simulink library "lib_IC_GFM"  (R2026a)
settings: Solver=VariableStepAuto
undefined symbols (not defined in the file): block_buses, block_buses_DC, block_idx, block_toM, buses_lf, fb, fref, iC, invL, iR, iTf, Kic, Kiv, Kpc, Kpv, Nbuses_DC, omegab, op_intconv_GFM
libraries: simulink x4, sl_discontinuities x2
(part 1 of 2)
settings Model: Creator=atomas  LastModifiedBy=atomas

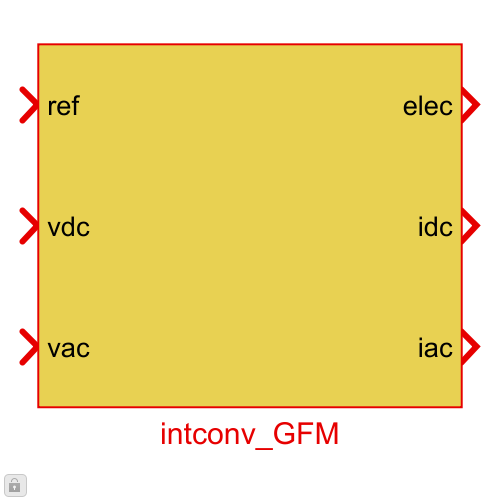
[thumbnail: Simulink's stored preview of the top-level diagram]
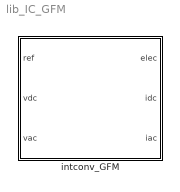
== system lib_IC_GFM ==
  intconv_GFM : Subsystem  mask(VCVSC){dynamic_VCC=Static, Lf=0.01, Rf=0.001, Rcf=1000000, Cfi=0.1, Kint=1, Tint=0.1, Bint=1, Kext=1, Bext=1, Text=0.1, Fi=1, Tf=0.01, mp=0.01, nq=0.01, VI_L=0.1, VI_R=0.01, WOF_Tf=0, L_out=0.1, R_out=0.01}
      mask prompts: dynamic_VCC "Dynamic behavior"; Lf "Filter inductance (pu)"; Rf "Filter resistance (pu)"; Rcf "Parallel resistance to C (pu)"; Cfi "Filter capacitance (pu)"; Fi "Current feedfordward gain"; Tf "Low-pass filter time constant (s)"; mp "Droop coefficient mp (pu)"; nq "Droop coefficient nq (pu)"; VI_L "Inductance (pu)"; VI_R "Resistance (pu)"; WOF_Tf "WOF time constant (s)"; L_out "Output inductance (p.u.)"; R_out "Output resistance (p.u.)"
      mask help: Grid-forming converter. VCC are the voltage and current controllers. Dynamic behavior includes the PI controllers, decoupling, current feedfordward and LC output filter. Static behavior consists of setting the reference voltage directly in the output. PC is the power controller including the droop control and low-pass filters for the power measurements.
      mask init:
      | [block_DC_buses, block_buses, block_DC_toM, block_toM, dparams, block_fref, block_idx, vcc_mode] = mask_init_intconv_GFM(gcb, dynamic_VCC);
      mask Help: web('Documentation/VCVSC.html')
      mask TypeOptions dynamic_VCC: Dynamic with limitation | Dynamic | Static | Dynamic VC and static CC
      mask TypeOptions Tf: PC/Tf
      mask TypeOptions mp: PC/mp
      mask TypeOptions nq: PC/nq
      mask TypeOptions VI_L: VI/L
      mask TypeOptions VI_R: VI/R
      mask TypeOptions WOF_Tf: VI/Tf
      mask DialogControl Container8 Prompt: Parameters
      mask DialogControl VCC Prompt: VCC
      mask DialogControl PC Prompt: PC
      mask DialogControl VI Prompt: VI
      mask DialogControl Container9 Prompt: Others

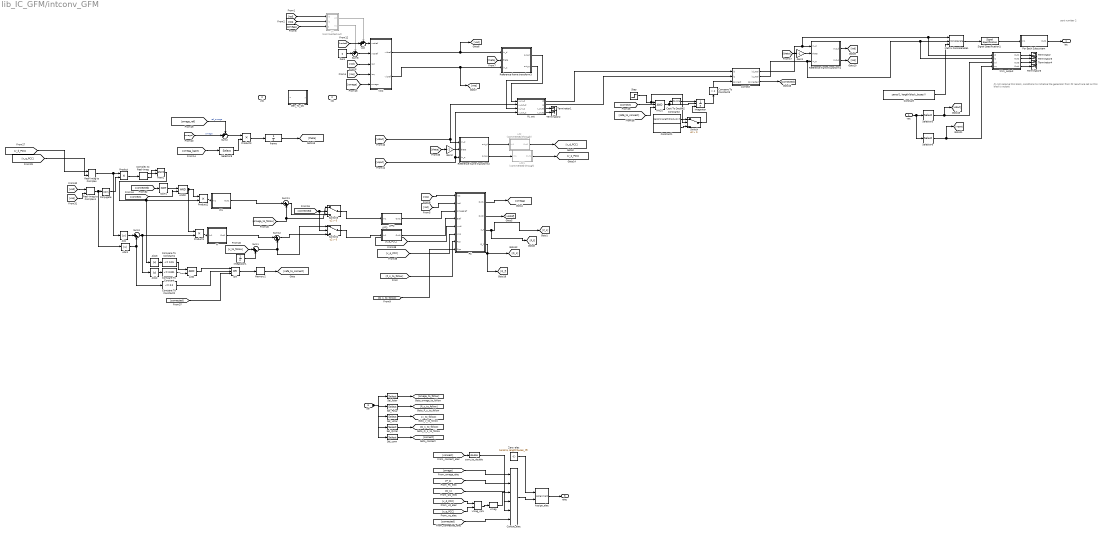
== system lib_IC_GFM/intconv_GFM ==
  note: port number 2
  note: do not rename this block, conditions to initialise the generator from PF result are set on this block's output
  vac : Inport
  vdc : Inport  Port=2
  ref : Inport  Port=3
  AND : Logic  IconShape=distinctive  AllPortsSameDT=off  OutDataTypeStr=boolean
  AND1 : Logic  Inputs=3  IconShape=distinctive  AllPortsSameDT=off  OutDataTypeStr=boolean
  AND2 : Logic  IconShape=distinctive  AllPortsSameDT=off  OutDataTypeStr=boolean
  Abs{,1..3} (4 alike) : Abs  ZeroCross=off  SaturateOnIntegerOverflow=off
  Assign_elec : Assignment  NumberOfDimensions=2  DiagnosticForDimensions=Warning  IndexOptions=Assign all,Index vector (dialog)  Indices=1,block_idx  OutputSizes=1
  Atan2 : Trigonometry  Operator=atan2
  Cast To Double2 : DataTypeConversion  OutDataTypeStr=double  SaturateOnIntegerOverflow=off  RndMeth=Floor
  Compare To Constant : simulink/Logic and Bit Operations/Compare To Constant  relop=<=  const=0.001  OutDataTypeStr=boolean  ZeroCross=off
  Compare To Constant1 : simulink/Logic and Bit Operations/Compare To Constant  relop=<=  const=0.01  OutDataTypeStr=boolean  ZeroCross=off
  Compare To Constant2 : simulink/Logic and Bit Operations/Compare To Constant  relop=<=  const=0.2  OutDataTypeStr=boolean  ZeroCross=off
  Compare To Constant3 : simulink/Logic and Bit Operations/Compare To Constant  relop=>  const=4  OutDataTypeStr=boolean  ZeroCross=off
  Complex to Real-Imag : ComplexToRealImag
  Concat_elec : Concatenate  NumInputs=6  Mode=Multidimensional array
  Conjugate : Math  Operator=conj  SignedPower=on  RndMeth=Zero
  Constant : Constant  Value=zeros(1, length(block_buses))  VectorParams1D=off
  Constant1 : Constant  Value=5*ones(1,length(block_idx))  VectorParams1D=off
  Constant2 : Constant  Value=zeros(1,length(block_idx))  VectorParams1D=off
  For Each Subsystem : Subsystem  TreatAsAtomicUnit=on
  Gain1 : Gain  Gain=-1
  Gain2 : Gain  Gain=-1
  Gen_To_DC : MATLAB Function  TreatAsAtomicUnit=on
  Integrator : Integrator  ExternalReset=falling  InitialConditionSource=external  InitialCondition=op_intconv_GFM.Integrator
  Integrator1 : Integrator  InitialCondition=op_intconv_GFM.Integrator1
  LPF : Subsystem  Commented=through
  LPF1 : Subsystem  Commented=through
  LPF2 : Subsystem
  LPF3 : Subsystem
  Matrix Concatenate1 : Concatenate  NumInputs=3  Mode=Multidimensional array
  Memory2 : Memory  InitialCondition=1
  NOT1 : Logic  Operator=NOT  IconShape=distinctive  AllPortsSameDT=off  OutDataTypeStr=boolean
  OR : Logic  Operator=OR  Inputs=3  IconShape=distinctive  AllPortsSameDT=off  OutDataTypeStr=boolean
  PC : Subsystem  mask(PC_VCVSC){Tf=Tf, mp=mp, nq=nq}
      mask prompts: Tf "Low-pass filter time constant (s)"; mp "Droop coefficient mp"; nq "Droop coefficient nq"
      mask help: Power controller of a grid-forming converter, including the droop control and low-pass filters for the power measurements.
      mask init:
      | [iTf, use_Tf] = mask_init_opt_filter(Tf);
  PI : Subsystem
  PI1 : Subsystem
  Product : Product
  Product1 : Product  OutDataTypeStr=double
  Product2 : Product  OutDataTypeStr=double
  Product3 : Product
  RL out : Subsystem  Variant=on  mask{dynamic=Dynamic, R=R_out, L=L_out, fbase=50}
      mask prompts: dynamic "Dynamic behavior"; R "Series resistance (p.u.)"; L "Inductance (p.u.)"; fbase "Base frequency (Hz)"
      mask init:
      | [invL, omegab, rl_mode] = mask_init_RL(dynamic, L, fbase);
      mask TypeOptions dynamic: Static | Dynamic | Static omega
  Real-Imag to Complex : RealImagToComplex
  Real-Imag to Complex1 : RealImagToComplex
  Reference frame transform1 : Subsystem
  Reference frame transform2 : Subsystem
  Reference frame transform3 : Subsystem
  Sel_Pstar : Selector  NumberOfDimensions=2  InputPortWidth=3  IndexOptions=Index vector (dialog),Index vector (dialog)  Indices=2,block_idx  OutputSizes=1
  Sel_Qstar : Selector  NumberOfDimensions=2  InputPortWidth=3  IndexOptions=Index vector (dialog),Index vector (dialog)  Indices=4,block_idx  OutputSizes=1
  Sel_conn : Selector  NumberOfDimensions=2  InputPortWidth=3  IndexOptions=Index vector (dialog),Index vector (dialog)  Indices=5,block_idx  OutputSizes=1
  Sel_fstar : Selector  NumberOfDimensions=2  InputPortWidth=3  IndexOptions=Index vector (dialog),Index vector (dialog)  Indices=1,block_idx  OutputSizes=1
  Sel_vstar : Selector  NumberOfDimensions=2  InputPortWidth=3  IndexOptions=Index vector (dialog),Index vector (dialog)  Indices=3,block_idx  OutputSizes=1
  Selector5 : Selector  NumberOfDimensions=2  InputPortWidth=3  IndexOptions=Index vector (dialog),Index vector (dialog)  Indices=1,block_buses  OutputSizes=1,1
  Selector6 : Selector  NumberOfDimensions=2  InputPortWidth=3  IndexOptions=Index vector (dialog),Index vector (dialog)  Indices=2,block_buses  OutputSizes=1,1
  Selector8 : Selector  InputPortWidth=length(fref.ref_units)  IndexOptions=Index vector (dialog)  Indices=block_fref  OutputSizes=1
  Signal Specification1 : SignalSpecification  Dimensions=[3 length(block_buses)]
  Step : Step  Time=0.01  SampleTime=0  VectorParams1D=off  ZeroCross=off
  Sum1 : Sum  Inputs=|++
  Sum11 : Sum  Inputs=|++
  Sum12 : Sum  Inputs=|++
  Sum2 : Sum  Inputs=-+|
  Sum3 : Sum  Inputs=|+-
  Sum8 : Sum  Inputs=++|
  Switch : Switch  Criteria=u2 > Threshold  SaturateOnIntegerOverflow=off  InputSameDT=off
  Switch2 : Switch  Criteria=u2 > Threshold  SaturateOnIntegerOverflow=off  InputSameDT=off
  Switch3 : Switch  Criteria=u2 > Threshold  SaturateOnIntegerOverflow=off  InputSameDT=off
  Terminator{,1..5} (6 alike) : Terminator
  VCC : Subsystem  Variant=on
  VI : Subsystem  Commented=on  mask{L=VI_L, R=VI_R, Tf=WOF_Tf}
      mask prompts: L "Inductance (pu)"; R "Resistance (pu)"; Tf "WOF time constant (s)"
      mask init:
      | [iTf, use_Tf] = mask_init_opt_filter(Tf);
  Zero : Constant  Value=0  OutDataTypeStr=Inherit: Inherit via back propagation
  Zero_elec : Constant  Value=zeros(6, length(buses_lf))
  conn_to_double : DataTypeConversion  OutDataTypeStr=double  SaturateOnIntegerOverflow=off  RndMeth=Floor
  connect : Subsystem
  frame : Integrator  InitialCondition=op_intconv_GFM.frame  IgnoreLimit=on
  trim_output : Subsystem
  vmag : ComplexToMagnitudeAngle  Output=Magnitude
  vmag_cplx : RealImagToComplex
  vod : Sum  Inputs=++|
  iac : Outport
  idc : Outport  Port=2
  elec : Outport  Port=3
  wires:
  LPF3/1(Out1) -> PC/4(Eref)
  LPF2/1(Out1) -> PC/3(omegaref)
  [connect] -> AND2/2
  Compare To Constant3/1 -> connect/3(connect)
  Integrator1/1 -> Sum1/2
  [v_to_follow] -> Sum1/1
  [Q_s_to_follow] -> PC/8(Qsp)
  [P_s_to_follow] -> PC/7(Psp)
  Switch2/1 -> LPF3/1(In1)
  Switch3/1 -> LPF2/1(In1)
  Sum11/1 -> Switch3/3
  PI1/1(Out1) -> Sum11/1
  PI/1(Out1) -> Sum12/1
  [connected] -> Switch3/2, Switch2/2
  [omega_to_follow] -> Switch3/1, Sum11/2
  Sum1/1 -> Sum12/2, Switch2/1
  Sum12/1 -> Switch2/3
  VCC/2(viqref) -> Reference frame transform3/3(in_q), [voq]
  VCC/1(vidref) -> Reference frame transform3/1(in_d), [vod]
  Switch/1 -> Integrator/3
  Cast To Double2/1 -> Integrator/1
  AND1/1 -> Integrator/2, Cast To Double2/1
  [safe_to_connect] -> AND1/3
  Constant1/1 -> Switch/3
  Step/1 -> AND1/1, Switch/2
  Constant2/1 -> Switch/1
  Integrator/1 -> Compare To Constant3/1
  [connect] -> AND1/2
  AND2/1 -> Product2/1, Product1/1
  [connected] -> NOT1/1
  NOT1/1 -> AND2/1
  Selector5/1 -> trim_output/3(vd), [vdout]
  Selector6/1 -> trim_output/4(vq), [vqout]
  vac/1 -> Selector5/1, Selector6/1
  trim_output/4(Out4) -> Terminator5/1
  trim_output/3(Out3) -> Terminator4/1
  trim_output/2(Out2) -> Terminator3/1
  trim_output/1(Out1) -> Terminator/1
  [v_q_PCC] -> PC/6(voq)
  [v_d_PCC] -> PC/5(vodi)
  Signal Specification1/1 -> For Each Subsystem/1(In1)
  For Each Subsystem/1(Out1) -> iac/1
  Constant/1 -> Matrix Concatenate1/3
  Matrix Concatenate1/1 -> Signal Specification1/1
  [vdout] -> Reference frame transform2/1(in_d), RL out/2(v_out_d)
  LPF1/1(Out1) -> [v_q_PCC]
  LPF/1(Out1) -> [v_d_PCC]
  [vqout] -> RL out/4(v_out_q), Reference frame transform2/3(in_q)
  Memory2/1 -> [safe_to_connect]
  [connected] -> OR/3
  Compare To Constant2/1 -> OR/2
  OR/1 -> Memory2/1
  AND/1 -> OR/1
  Compare To Constant1/1 -> AND/1
  Abs3/1 -> Compare To Constant1/1
  Compare To Constant/1 -> AND/2
  Abs2/1 -> Compare To Constant/1
  Abs1/1 -> Sum3/2, Compare To Constant2/1
  Atan2/1 -> Product2/2, Abs3/1
  Product2/1 -> PI1/1(In1)
  Product1/1 -> PI/1(In1)
  Sum3/1 -> Product1/2, Abs2/1
  Abs/1 -> Sum3/1
  Complex to Real-Imag/1 -> Atan2/2
  Complex to Real-Imag/2 -> Atan2/1
  Product/1 -> Complex to Real-Imag/1
  Conjugate/1 -> Product/2
  Real-Imag to Complex/1 -> Product/1, Abs/1
  Real-Imag to Complex1/1 -> Conjugate/1, Abs1/1
  [voq] -> Real-Imag to Complex1/2
  [vod] -> Real-Imag to Complex1/1
  [v_q_PCC] -> Real-Imag to Complex/2
  [v_d_PCC] -> Real-Imag to Complex/1
  Reference frame transform2/2(out_q) -> LPF1/1(In1)
  Reference frame transform2/1(out_d) -> LPF/1(In1)
  RL out/4(v_outq) -> Terminator2/1
  RL out/3(v_outd) -> Terminator1/1
  connect/2(iq_real) -> Reference frame transform1/3(in_q), Matrix Concatenate1/2, trim_output/2(iq)
  connect/1(id_real) -> Reference frame transform1/1(in_d), Matrix Concatenate1/1, trim_output/1(id)
  VI/2(vq) -> Sum8/1
  VI/1(vd) -> vod/1
  Reference frame transform1/1(out_d) -> [iod]
  RL out/2(iq) -> connect/2(iq)
  Reference frame transform3/2(out_q) -> RL out/3(v_in_q)
  Reference frame transform3/1(out_d) -> RL out/1(v_in_d)
  Reference frame transform1/2(out_q) -> [ioq]
  [ioq] -> PC/1(ioq)
  [iod] -> PC/2(iodi)
  PC/2(Out2) -> [vodref]
  PC/1(Out1) -> [omega]
  [theta] -> Reference frame transform3/2(theta)
  [omega] -> VCC/5(omega)
  [vodref] -> vod/2
  Zero/1 -> Sum8/2
  [iod] -> VCC/3(iod)
  [ioq] -> VCC/4(ioq)
  Gain1/1 -> Reference frame transform1/2(theta)
  [theta] -> Gain1/1
  RL out/1(id) -> connect/1(id)
  Sum2/1 -> Product3/1
  [omega_ref] -> Sum2/1  "ref_omega"
  [omega] -> Sum2/2  "omega"
  connect/3(connected) -> [connected]
  PC/3(P_f) -> [P_f], [P_s]
  PC/4(Q_f) -> [Q_f], [Q_s]
  frame/1 -> [theta]
  Product3/1 -> frame/1
  [theta] -> Gain2/1
  Gain2/1 -> Reference frame transform2/2(theta)
  [iod] -> VI/1(id)
  [ioq] -> VI/2(iq)
  [omega] -> VI/3(omega)
  vod/1 -> VCC/1(vodref)
  Sum8/1 -> VCC/2(voqref)
  Selector8/1 -> Product3/2
  [omega_base] -> Selector8/1
  ref/1 -> Sel_fstar/1, Sel_Pstar/1, Sel_vstar/1, Sel_Qstar/1, Sel_conn/1
  Sel_fstar/1 -> [omega_to_follow]
  Sel_Pstar/1 -> [P_s_to_follow]
  Sel_vstar/1 -> [v_to_follow]
  Sel_Qstar/1 -> [Q_s_to_follow]
  Sel_conn/1 -> [connect]
  [connect] -> conn_to_double/1
  [v_d_PCC] -> vmag_cplx/1
  [v_q_PCC] -> vmag_cplx/2
  vmag_cplx/1 -> vmag/1
  [omega] -> Concat_elec/1
  [P_s] -> Concat_elec/2
  vmag/1 -> Concat_elec/3
  [Q_s] -> Concat_elec/4
  conn_to_double/1 -> Concat_elec/5
  [connected] -> Concat_elec/6
  Zero_elec/1 -> Assign_elec/1
  Concat_elec/1 -> Assign_elec/2
  Assign_elec/1 -> elec/1

== system lib_IC_GFM/intconv_GFM/For Each Subsystem ==
  In1 : Inport  Partition=on  PartitionDimension=1  PartitionWidth=1  PartitionOffset=0
  For Each : ForEach  DisableCoverage=on
  State-Space : StateSpace  A=[]  B=[]  C=[]  D=block_toM  InitialCondition=0  ParameterTunability=Optimized
  Transpose : Math  Operator=transpose
  Transpose1 : Math  Operator=transpose
  Out1 : Outport  ConcatenationDimension=1
  wires:
  In1/1 -> Transpose/1
  Transpose1/1 -> Out1/1
  Transpose/1 -> State-Space/1
  State-Space/1 -> Transpose1/1

== system lib_IC_GFM/intconv_GFM/LPF ==
  In1 : Inport
  Gain : Gain  Gain=1e2
  I : Integrator  InitialCondition=op_intconv_GFM.LPF_I
  Sum4 : Sum  Inputs=|+-
  Out1 : Outport
  wires:
  I/1 -> Sum4/2, Out1/1
  In1/1 -> Sum4/1
  Sum4/1 -> Gain/1
  Gain/1 -> I/1

== system lib_IC_GFM/intconv_GFM/LPF1 ==
  In1 : Inport
  Gain : Gain  Gain=1e2
  I : Integrator  InitialCondition=op_intconv_GFM.LPF1_I
  Sum4 : Sum  Inputs=|+-
  Out1 : Outport
  wires:
  Gain/1 -> I/1
  Sum4/1 -> Gain/1
  In1/1 -> Sum4/1
  I/1 -> Out1/1, Sum4/2

== system lib_IC_GFM/intconv_GFM/LPF2 ==
  In1 : Inport
  Gain : Gain  Gain=1e2
  I : Integrator  InitialCondition=op_intconv_GFM.LPF2_I
  Sum4 : Sum  Inputs=|+-
  Out1 : Outport
  wires:
  Gain/1 -> I/1
  Sum4/1 -> Gain/1
  In1/1 -> Sum4/1
  I/1 -> Out1/1, Sum4/2

== system lib_IC_GFM/intconv_GFM/LPF3 ==
  In1 : Inport
  Gain : Gain  Gain=1e2
  I : Integrator  InitialCondition=op_intconv_GFM.LPF3_I
  Sum4 : Sum  Inputs=|+-
  Out1 : Outport
  wires:
  I/1 -> Sum4/2, Out1/1
  In1/1 -> Sum4/1
  Sum4/1 -> Gain/1
  Gain/1 -> I/1

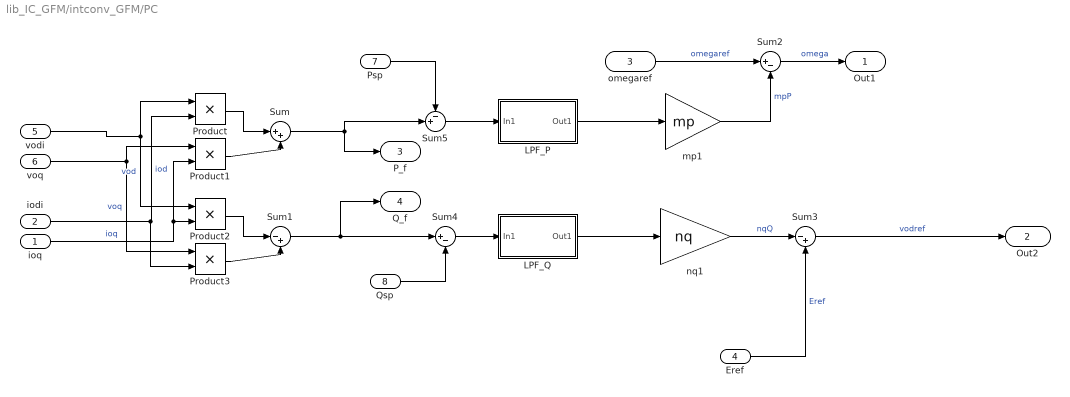
== system lib_IC_GFM/intconv_GFM/PC ==
  ioq : Inport
  iodi : Inport  Port=2
  omegaref : Inport  Port=3
  Eref : Inport  Port=4
  vodi : Inport  Port=5
  voq : Inport  Port=6
  Psp : Inport  Port=7
  Qsp : Inport  Port=8
  LPF_P : Subsystem  Variant=on
  LPF_Q : Subsystem  Variant=on
  Product{,1..3} (4 alike) : Product
  Sum : Sum  Inputs=|++
  Sum1 : Sum  Inputs=|-+
  Sum2 : Sum  Inputs=|+-
  Sum3 : Sum  Inputs=|-+
  Sum4 : Sum  Inputs=|+-
  Sum5 : Sum  Inputs=-+|
  mp1 : Gain  Gain=mp
  nq1 : Gain  Gain=nq
  Out1 : Outport
  Out2 : Outport  Port=2
  P_f : Outport  Port=3
  Q_f : Outport  Port=4
  wires:
  LPF_Q/1(Out1) -> nq1/1
  Sum4/1 -> LPF_Q/1(In1)
  LPF_P/1(Out1) -> mp1/1
  Sum5/1 -> LPF_P/1(In1)
  Sum3/1 -> Out2/1  "vodref"
  Psp/1 -> Sum5/1
  Qsp/1 -> Sum4/2
  ioq/1 -> Product1/2, Product2/2  "ioq"
  iodi/1 -> Product/2, Product3/2  "iod"
  voq/1 -> Product3/1, Product1/1  "voq"
  mp1/1 -> Sum2/2  "mpP"
  Sum1/1 -> Sum4/1, Q_f/1
  Sum/1 -> P_f/1, Sum5/2
  omegaref/1 -> Sum2/1  "omegaref"
  Eref/1 -> Sum3/2  "Eref"
  nq1/1 -> Sum3/1  "nqQ"
  Product3/1 -> Sum1/2
  Product2/1 -> Sum1/1
  Product1/1 -> Sum/2
  Product/1 -> Sum/1
  vodi/1 -> Product/1, Product2/1  "vod"
  Sum2/1 -> Out1/1  "omega"

== system lib_IC_GFM/intconv_GFM/PI ==
  In1 : Inport
  Gain : Gain  Gain=0.1
  Gain1 : Gain  Gain=0.2
  I : Integrator  InitialCondition=op_intconv_GFM.PI_I
  Sum10 : Sum  Inputs=|++
  Out1 : Outport
  wires:
  In1/1 -> Gain1/1, Gain/1
  Sum10/1 -> Out1/1
  Gain/1 -> Sum10/1
  I/1 -> Sum10/2
  Gain1/1 -> I/1

== system lib_IC_GFM/intconv_GFM/PI1 ==
  In1 : Inport
  Gain : Gain  Gain=0.1/100/pi
  Gain1 : Gain  Gain=0.2/100/pi
  I : Integrator  InitialCondition=op_intconv_GFM.PI1_I
  Sum10 : Sum  Inputs=|++
  Out1 : Outport
  wires:
  Gain1/1 -> I/1
  I/1 -> Sum10/2
  Gain/1 -> Sum10/1
  Sum10/1 -> Out1/1
  In1/1 -> Gain/1, Gain1/1

== system lib_IC_GFM/intconv_GFM/RL out ==
  note: 1) Add Subsystem or Model blocks as valid variant choices.
      | 2) You cannot connect blocks at this level. At simulation, connectivity is automatically
      | determined, based on the active variant and port name matching.
  v_in_d : Inport
  v_out_d : Inport  Port=2
  v_in_q : Inport  Port=3
  v_out_q : Inport  Port=4
  dynamic : Subsystem  VariantControl=rl_mode == 1
  static : Subsystem  VariantControl=rl_mode == 2
  static_omega : Subsystem  VariantControl=(default)
  id : Outport
  iq : Outport  Port=2
  v_outd : Outport  Port=3
  v_outq : Outport  Port=4

== system lib_IC_GFM/intconv_GFM/Reference frame transform1 ==
  in_d : Inport
  theta : Inport  Port=2
  in_q : Inport  Port=3
  Complex to Real-Imag : ComplexToRealImag
  Cos : Trigonometry  SCDEnableBlockLinearizationSpecification=on  Operator=cos
  Product : Product
  Real-Imag to Complex : RealImagToComplex
  Real-Imag to Complex1 : RealImagToComplex
  Sin : Trigonometry  SCDEnableBlockLinearizationSpecification=on
  out_d : Outport
  out_q : Outport  Port=2
  wires:
  in_d/1 -> Real-Imag to Complex/1
  in_q/1 -> Real-Imag to Complex/2
  Complex to Real-Imag/1 -> out_d/1
  Sin/1 -> Real-Imag to Complex1/2
  Cos/1 -> Real-Imag to Complex1/1
  theta/1 -> Cos/1, Sin/1
  Product/1 -> Complex to Real-Imag/1
  Real-Imag to Complex/1 -> Product/2
  Real-Imag to Complex1/1 -> Product/1
  Complex to Real-Imag/2 -> out_q/1

== system lib_IC_GFM/intconv_GFM/Reference frame transform2 ==
  in_d : Inport
  theta : Inport  Port=2
  in_q : Inport  Port=3
  Complex to Real-Imag : ComplexToRealImag
  Cos : Trigonometry  SCDEnableBlockLinearizationSpecification=on  Operator=cos
  Product : Product
  Real-Imag to Complex : RealImagToComplex
  Real-Imag to Complex1 : RealImagToComplex
  Sin : Trigonometry  SCDEnableBlockLinearizationSpecification=on
  out_d : Outport
  out_q : Outport  Port=2
  wires:
  Complex to Real-Imag/2 -> out_q/1
  Real-Imag to Complex1/1 -> Product/1
  Real-Imag to Complex/1 -> Product/2
  Product/1 -> Complex to Real-Imag/1
  theta/1 -> Sin/1, Cos/1
  Cos/1 -> Real-Imag to Complex1/1
  Sin/1 -> Real-Imag to Complex1/2
  Complex to Real-Imag/1 -> out_d/1
  in_q/1 -> Real-Imag to Complex/2
  in_d/1 -> Real-Imag to Complex/1

== system lib_IC_GFM/intconv_GFM/Reference frame transform3 ==
  in_d : Inport
  theta : Inport  Port=2
  in_q : Inport  Port=3
  Complex to Real-Imag : ComplexToRealImag
  Cos : Trigonometry  SCDEnableBlockLinearizationSpecification=on  Operator=cos
  Product : Product
  Real-Imag to Complex : RealImagToComplex
  Real-Imag to Complex1 : RealImagToComplex
  Sin : Trigonometry  SCDEnableBlockLinearizationSpecification=on
  out_d : Outport
  out_q : Outport  Port=2
  wires:
  in_d/1 -> Real-Imag to Complex/1
  in_q/1 -> Real-Imag to Complex/2
  Complex to Real-Imag/1 -> out_d/1
  Sin/1 -> Real-Imag to Complex1/2
  Cos/1 -> Real-Imag to Complex1/1
  theta/1 -> Sin/1, Cos/1
  Product/1 -> Complex to Real-Imag/1
  Real-Imag to Complex/1 -> Product/2
  Real-Imag to Complex1/1 -> Product/1
  Complex to Real-Imag/2 -> out_q/1

== system lib_IC_GFM/intconv_GFM/VCC ==
  note: 1) Add Subsystem or Model blocks as valid variant choices.
      | 2) You cannot connect blocks at this level. At simulation, connectivity is automatically
      | determined, based on the active variant and port name matching.
  vodref : Inport
  voqref : Inport  Port=2
  iod : Inport  Port=3
  ioq : Inport  Port=4
  omega : Inport  Port=5
  dynamic : Subsystem  VariantControl=vcc_mode == 1
  dynamic_VC : Subsystem  VariantControl=vcc_mode == 3
  dynamic_limiting : Subsystem  VariantControl=vcc_mode == 2
  static : Subsystem  VariantControl=(default)
  vidref : Outport
  viqref : Outport  Port=2

== system lib_IC_GFM/intconv_GFM/VI ==
  id : Inport
  iq : Inport  Port=2
  omega : Inport  Port=3
  Gain : Gain  Gain=L
  Gain1 : Gain  Gain=R
  Gain2 : Gain  Gain=L
  Gain3 : Gain  Gain=R
  Product : Product
  Product1 : Product
  Sum : Sum  Inputs=-+|
  Sum1 : Sum  Inputs=|--
  WOF_d : Subsystem  Variant=on
  WOF_q : Subsystem  Variant=on
  vd : Outport
  vq : Outport  Port=2
  wires:
  WOF_q/1(Out1) -> Gain3/1, Gain/1
  iq/1 -> WOF_q/1(In1)
  WOF_d/1(Out1) -> Gain2/1, Gain1/1
  id/1 -> WOF_d/1(In1)
  Gain/1 -> Product/1
  omega/1 -> Product/2, Product1/1
  Product/1 -> Sum/2
  Gain2/1 -> Product1/2
  Product1/1 -> Sum1/1
  Gain1/1 -> Sum/1
  Gain3/1 -> Sum1/2
  Sum/1 -> vd/1
  Sum1/1 -> vq/1

== system lib_IC_GFM/intconv_GFM/connect ==
  id : Inport
  iq : Inport  Port=2
  connect : Inport  Port=3
  Switch : Switch  Criteria=u2 > Threshold  ZeroCross=off  SaturateOnIntegerOverflow=off  InputSameDT=off
  Switch1 : Switch  Criteria=u2 > Threshold  ZeroCross=off  SaturateOnIntegerOverflow=off  InputSameDT=off
  Zero1 : Constant  Value=0  VectorParams1D=off  OutDataTypeStr=Inherit: Inherit via back propagation
  Zero2 : Constant  Value=0  VectorParams1D=off  OutDataTypeStr=Inherit: Inherit via back propagation
  id_real : Outport
  iq_real : Outport  Port=2
  connected : Outport  Port=3  OutDataTypeStr=boolean
  wires:
  Zero2/1 -> Switch1/3
  iq/1 -> Switch1/1
  Switch1/1 -> iq_real/1
  connect/1 -> Switch/2, Switch1/2, connected/1
  id/1 -> Switch/1
  Zero1/1 -> Switch/3
  Switch/1 -> id_real/1

== system lib_IC_GFM/intconv_GFM/trim_output ==
  id : Inport
  iq : Inport  Port=2
  vd : Inport  Port=3
  vq : Inport  Port=4
  Out1 : Outport
  Out2 : Outport  Port=2
  Out3 : Outport  Port=3
  Out4 : Outport  Port=4
  wires:
  iq/1 -> Out2/1
  vd/1 -> Out3/1
  vq/1 -> Out4/1
  id/1 -> Out1/1

== system lib_IC_GFM/intconv_GFM/PC/LPF_P ==
  note: 1) Add Subsystem or Model blocks as valid variant choices.
      | 2) You cannot connect blocks at this level. At simulation, connectivity is automatically
      | determined, based on the active variant and port name matching.
  In1 : Inport
  Active : Subsystem  VariantControl=use_Tf == 1
  Bypass : Subsystem  VariantControl=(default)
  Out1 : Outport

== system lib_IC_GFM/intconv_GFM/PC/LPF_Q ==
  note: 1) Add Subsystem or Model blocks as valid variant choices.
      | 2) You cannot connect blocks at this level. At simulation, connectivity is automatically
      | determined, based on the active variant and port name matching.
  In1 : Inport
  Active : Subsystem  VariantControl=use_Tf == 1
  Bypass : Subsystem  VariantControl=(default)
  Out1 : Outport

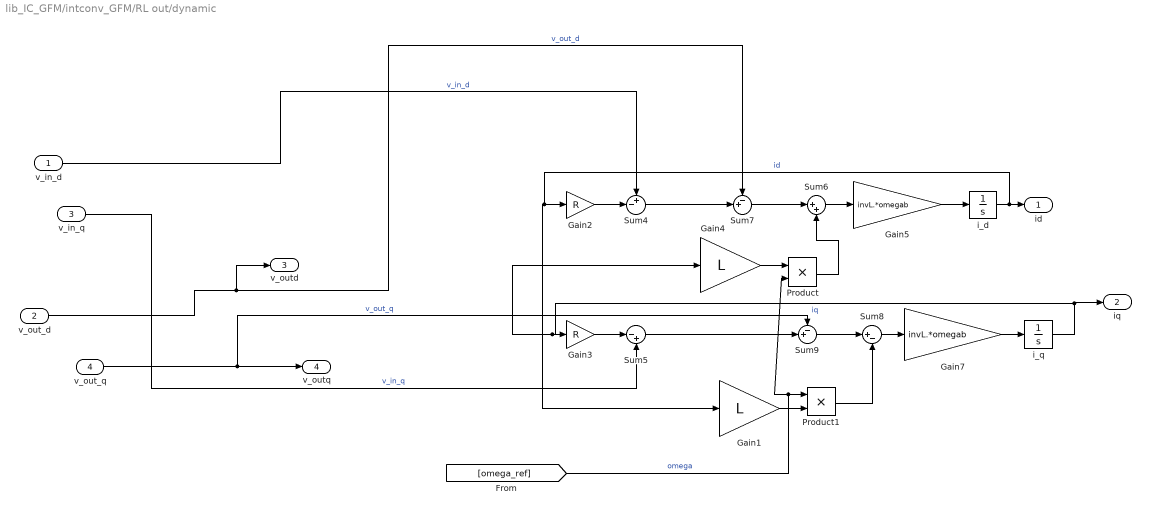
== system lib_IC_GFM/intconv_GFM/RL out/dynamic ==
  v_in_d : Inport
  v_out_d : Inport  Port=2
  v_in_q : Inport  Port=3
  v_out_q : Inport  Port=4
  Gain1 : Gain  Gain=L
  Gain2 : Gain  Gain=R
  Gain3 : Gain  Gain=R
  Gain4 : Gain  Gain=L
  Gain5 : Gain  Gain=invL.*omegab
  Gain7 : Gain  Gain=invL.*omegab
  Product : Product
  Product1 : Product
  Sum4 : Sum  Inputs=+-|
  Sum5 : Sum  Inputs=|-+
  Sum6 : Sum  Inputs=|++
  Sum7 : Sum  Inputs=-+|
  Sum8 : Sum  Inputs=|+-
  Sum9 : Sum  Inputs=-+|
  i_d : Integrator  InitialCondition=op_intconv_GFM.RL_out_dynamic_i_d
  i_q : Integrator  InitialCondition=op_intconv_GFM.RL_out_dynamic_i_q
  id : Outport
  iq : Outport  Port=2
  v_outd : Outport  Port=3
  v_outq : Outport  Port=4
  wires:
  v_in_q/1 -> Sum5/2  "v_in_q"
  v_in_d/1 -> Sum4/1  "v_in_d"
  Gain2/1 -> Sum4/2
  i_d/1 -> Gain2/1, Gain1/1, id/1  "id"
  Sum6/1 -> Gain5/1
  [omega_ref] -> Product1/1, Product/2  "omega"
  Gain5/1 -> i_d/1
  Product/1 -> Sum6/2
  Sum8/1 -> Gain7/1
  Sum4/1 -> Sum7/2
  Product1/1 -> Sum8/2
  Gain4/1 -> Product/1
  Sum7/1 -> Sum6/1
  Gain3/1 -> Sum5/1
  Sum5/1 -> Sum9/2
  Gain7/1 -> i_q/1
  i_q/1 -> Gain3/1, Gain4/1, iq/1  "iq"
  Gain1/1 -> Product1/2
  Sum9/1 -> Sum8/1
  v_out_d/1 -> Sum7/1, v_outd/1  "v_out_d"
  v_out_q/1 -> Sum9/1, v_outq/1  "v_out_q"

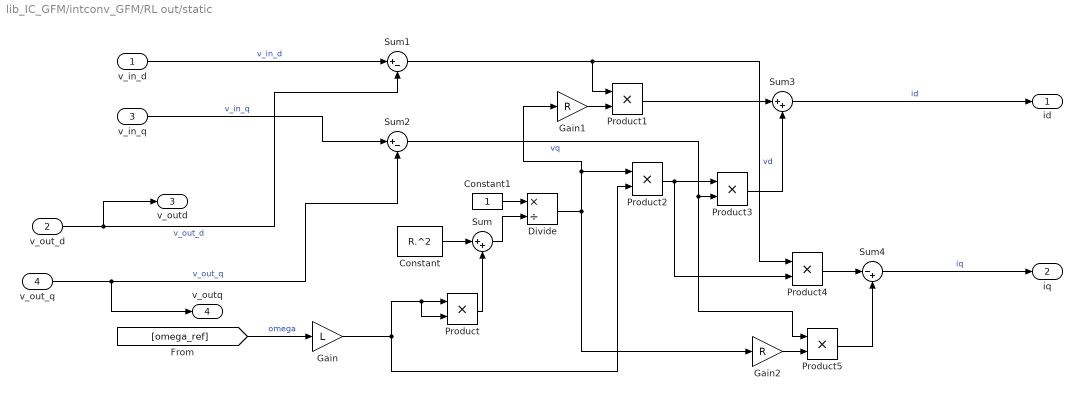
== system lib_IC_GFM/intconv_GFM/RL out/static ==
  v_in_d : Inport
  v_out_d : Inport  Port=2
  v_in_q : Inport  Port=3
  v_out_q : Inport  Port=4
  Constant : Constant  Value=R.^2
  Constant1 : Constant
  Divide : Product  Inputs=*/
  Gain : Gain  Gain=L
  Gain1 : Gain  Gain=R
  Gain2 : Gain  Gain=R
  Product{,1..5} (6 alike) : Product
  Sum : Sum  Inputs=|++
  Sum1 : Sum  Inputs=|+-
  Sum2 : Sum  Inputs=|+-
  Sum3 : Sum  Inputs=|++
  Sum4 : Sum  Inputs=|-+
  id : Outport
  iq : Outport  Port=2
  v_outd : Outport  Port=3
  v_outq : Outport  Port=4
  wires:
  v_in_q/1 -> Sum2/1  "v_in_q"
  v_out_d/1 -> Sum1/2, v_outd/1  "v_out_d"
  Sum/1 -> Divide/2
  Gain2/1 -> Product5/2
  Product/1 -> Sum/2
  Product1/1 -> Sum3/1
  Product5/1 -> Sum4/2
  Constant/1 -> Sum/1
  Sum2/1 -> Product3/2, Product5/1  "vq"
  Gain/1 -> Product2/2, Product/1, Product/2
  Constant1/1 -> Divide/1
  Product3/1 -> Sum3/2
  Sum1/1 -> Product4/1, Product1/1  "vd"
  Divide/1 -> Product2/1, Gain1/1, Gain2/1
  Product4/1 -> Sum4/1
  Product2/1 -> Product3/1, Product4/2
  Gain1/1 -> Product1/2
  Sum3/1 -> id/1  "id"
  Sum4/1 -> iq/1  "iq"
  v_out_q/1 -> Sum2/2, v_outq/1  "v_out_q"
  v_in_d/1 -> Sum1/1  "v_in_d"
  [omega_ref] -> Gain/1  "omega"

== system lib_IC_GFM/intconv_GFM/RL out/static_omega ==
  v_in_d : Inport
  v_out_d : Inport  Port=2
  v_in_q : Inport  Port=3
  v_out_q : Inport  Port=4
  Gain : Gain  Gain=1./(R.^2+L.^2)
  Gain2 : Gain  Gain=1./(R.^2+L.^2)
  Gain3 : Gain  Gain=R
  Gain4 : Gain  Gain=L
  Gain5 : Gain  Gain=L
  Gain6 : Gain  Gain=R
  Sum : Sum  Inputs=|++
  Sum1 : Sum  Inputs=|+-
  Sum2 : Sum  Inputs=|+-
  Sum3 : Sum  Inputs=|-+
  id : Outport
  iq : Outport  Port=2
  v_outd : Outport  Port=3
  v_outq : Outport  Port=4
  wires:
  Gain6/1 -> Sum3/2
  Sum3/1 -> iq/1
  Gain5/1 -> Sum3/1
  Sum/1 -> id/1
  Gain2/1 -> Gain4/1, Gain6/1
  Gain4/1 -> Sum/2
  Gain3/1 -> Sum/1
  Gain/1 -> Gain3/1, Gain5/1
  Sum2/1 -> Gain2/1  "vq"
  Sum1/1 -> Gain/1  "vd"
  v_out_d/1 -> Sum1/2, v_outd/1  "v_out_d"
  v_out_q/1 -> Sum2/2, v_outq/1  "v_out_q"
  v_in_d/1 -> Sum1/1  "v_in_d"
  v_in_q/1 -> Sum2/1  "v_in_q"

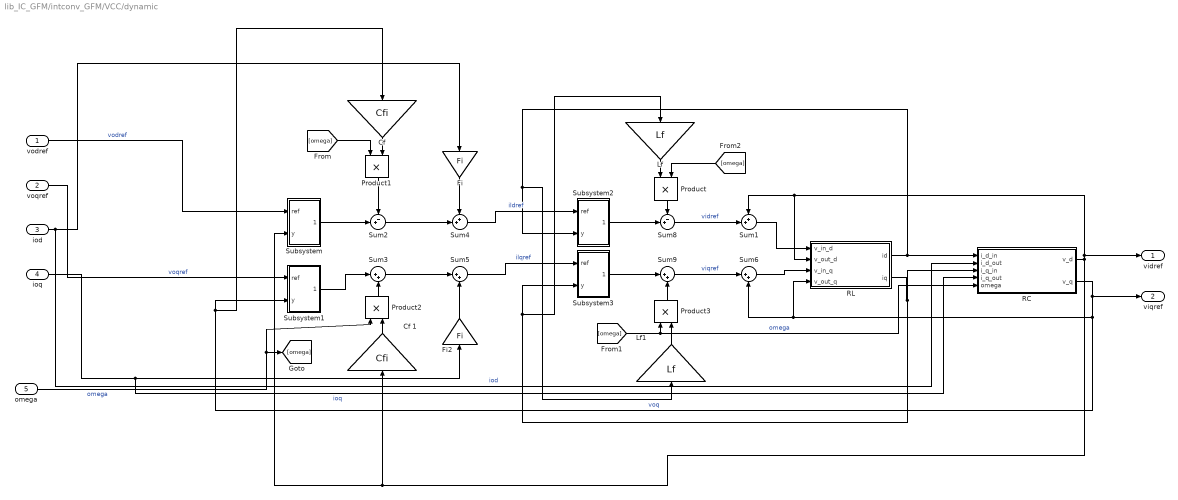
== system lib_IC_GFM/intconv_GFM/VCC/dynamic ==
  vodref : Inport
  voqref : Inport  Port=2
  iod : Inport  Port=3
  ioq : Inport  Port=4
  omega : Inport  Port=5
  Cf : Gain  Gain=Cfi
  Cf 1 : Gain  Gain=Cfi
  Fi : Gain  Gain=Fi
  Fi2 : Gain  Gain=Fi
  "Lf " : Gain  Gain=Lf
  Lf1 : Gain  Gain=Lf
  Product{,1..3} (4 alike) : Product
  RC : Subsystem  Variant=on  mask{dynamic=Dynamic, R=Rcf, C=Cfi, fbase=50}
      mask prompts: dynamic "Dynamic behavior"; R "Parallel resistance (p.u.)"; C "Capacitance (p.u.)"; fbase "Base frequency (Hz)"
      mask init:
      | [iC, iR, omegab, rc_mode] = mask_init_RC(dynamic, R, C, fbase);
      mask TypeOptions dynamic: Dynamic | Static | Static omega
  RL : Subsystem  Variant=on  mask(Line){dynamic=Dynamic, R=Rf, L=Lf, fbase=fb}
      mask prompts: dynamic "Dynamic behavior"; R "Series resistance (p.u.)"; L "Inductance (p.u.)"; fbase "Base frequency (Hz)"
      mask init:
      | [invL, omegab, rl_mode] = mask_init_RL(dynamic, L, fbase);
      mask Help: web('Documentation/RL.html')
      mask TypeOptions dynamic: Static | Dynamic | Static omega
  Subsystem : Subsystem
  Subsystem1 : Subsystem
  Subsystem2 : Subsystem
  Subsystem3 : Subsystem
  Sum1 : Sum  Inputs=++|
  Sum2 : Sum  Inputs=-+|
  Sum{3,5..6,9} (4 alike) : Sum  Inputs=|++
  Sum4 : Sum  Inputs=++|
  Sum8 : Sum  Inputs=-+|
  vidref : Outport
  viqref : Outport  Port=2
  wires:
  Sum6/1 -> RL/3(v_in_q)
  Sum1/1 -> RL/1(v_in_d)
  Sum9/1 -> Sum6/1  "viqref"
  Sum8/1 -> Sum1/2  "vidref"
  RL/2(iq) -> "Lf "/1, Subsystem3/2(y), RC/3(i_q_in)
  RL/1(id) -> RC/1(i_d_in), Lf1/1, Subsystem2/2(y)
  RC/1(v_d) -> Cf 1/1, Subsystem/2(y), RL/2(v_out_d), Sum1/1, vidref/1
  [omega] -> Product1/1
  omega/1 -> [omega], Product2/1  "omega"
  Subsystem3/1(Out1) -> Sum9/1
  Subsystem2/1(Out1) -> Sum8/2
  Subsystem1/1(Out1) -> Sum3/1
  Subsystem/1(Out1) -> Sum2/2
  Fi2/1 -> Sum5/2
  ioq/1 -> Fi2/1, RC/4(i_q_out)  "ioq"
  [omega] -> Product3/1, RC/5(omega)  "omega"
  Sum3/1 -> Sum5/1
  "Lf "/1 -> Product/1
  Sum2/1 -> Sum4/2
  iod/1 -> Fi/1, RC/2(i_d_out)  "iod"
  Product1/1 -> Sum2/1
  Sum4/1 -> Subsystem2/1(ref)  "ildref"
  Cf/1 -> Product1/2
  Cf 1/1 -> Product2/2
  Product2/1 -> Sum3/2
  Product3/1 -> Sum9/2
  voqref/1 -> Subsystem1/1(ref)  "voqref"
  Fi/1 -> Sum4/1
  Lf1/1 -> Product3/2
  [omega] -> Product/2
  RC/2(v_q) -> Cf/1, Subsystem1/2(y), RL/4(v_out_q), Sum6/2, viqref/1  "voq"
  vodref/1 -> Subsystem/1(ref)  "vodref"
  Product/1 -> Sum8/1
  Sum5/1 -> Subsystem3/1(ref)  "ilqref"

== system lib_IC_GFM/intconv_GFM/VCC/dynamic_VC ==
  vodref : Inport
  voqref : Inport  Port=2
  iod : Inport  Port=3
  ioq : Inport  Port=4
  omega : Inport  Port=5
  Cf : Gain  Gain=Cfi
  Cf 1 : Gain  Gain=Cfi
  Fi : Gain  Gain=Fi
  Fi2 : Gain  Gain=Fi
  Product1 : Product
  Product2 : Product
  RC : Subsystem  Variant=on  mask{dynamic=Dynamic, R=Rcf, C=Cfi, fbase=50}
      mask prompts: dynamic "Dynamic behavior"; R "Parallel resistance (p.u.)"; C "Capacitance (p.u.)"; fbase "Base frequency (Hz)"
      mask init:
      | [iC, iR, omegab, rc_mode] = mask_init_RC(dynamic, R, C, fbase);
      mask TypeOptions dynamic: Dynamic | Static | Static omega
  Subsystem : Subsystem
  Subsystem1 : Subsystem
  Sum2 : Sum  Inputs=-+|
  Sum3 : Sum  Inputs=|++
  Sum4 : Sum  Inputs=++|
  Sum5 : Sum  Inputs=|++
  vidref : Outport
  viqref : Outport  Port=2
  wires:
  Sum5/1 -> RC/3(i_q_in)
  Sum4/1 -> RC/1(i_d_in)
  RC/1(v_d) -> Subsystem/2(y), Cf 1/1, vidref/1
  vodref/1 -> Subsystem/1(ref)  "vodref"
  RC/2(v_q) -> Subsystem1/2(y), Cf/1, viqref/1
  Fi/1 -> Sum4/1
  voqref/1 -> Subsystem1/1(ref)  "voqref"
  Product2/1 -> Sum3/2
  Cf 1/1 -> Product2/2
  Cf/1 -> Product1/2
  Product1/1 -> Sum2/1
  iod/1 -> Fi/1, RC/2(i_d_out)  "iod"
  Sum2/1 -> Sum4/2
  Sum3/1 -> Sum5/1
  ioq/1 -> Fi2/1, RC/4(i_q_out)  "ioq"
  Fi2/1 -> Sum5/2
  Subsystem/1(Out1) -> Sum2/2
  Subsystem1/1(Out1) -> Sum3/1
  omega/1 -> [omega], Product2/1, RC/5(omega)  "omega"
  [omega] -> Product1/1

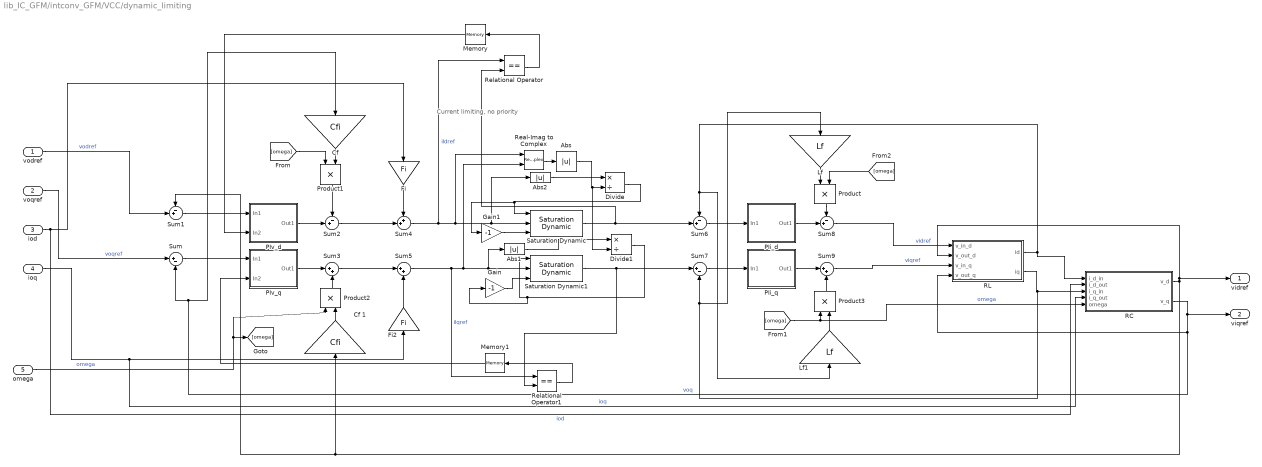
== system lib_IC_GFM/intconv_GFM/VCC/dynamic_limiting ==
  note: Current limiting, no priority
  vodref : Inport
  voqref : Inport  Port=2
  iod : Inport  Port=3
  ioq : Inport  Port=4
  omega : Inport  Port=5
  Abs : Abs  ZeroCross=off  SaturateOnIntegerOverflow=off
  Abs1 : Abs  ZeroCross=off  SaturateOnIntegerOverflow=off
  Abs2 : Abs  ZeroCross=off  SaturateOnIntegerOverflow=off
  Cf : Gain  Gain=Cfi
  Cf 1 : Gain  Gain=Cfi
  Divide : Product  Inputs=*/
  Divide1 : Product  Inputs=*/
  Fi : Gain  Gain=Fi
  Fi2 : Gain  Gain=Fi
  Gain : Gain  Gain=-1
  Gain1 : Gain  Gain=-1
  "Lf " : Gain  Gain=Lf
  Lf1 : Gain  Gain=Lf
  Memory : Memory  InitialCondition=1  LinearizeMemory=on
  Memory1 : Memory  InitialCondition=1  LinearizeMemory=on
  PIi_d : Subsystem
  PIi_q : Subsystem
  PIv_d : Subsystem
  PIv_q : Subsystem
  Product{,1..3} (4 alike) : Product
  RC : Subsystem  Variant=on  mask{dynamic=Dynamic, R=Rcf, C=Cfi, fbase=50}
      mask prompts: dynamic "Dynamic behavior"; R "Parallel resistance (p.u.)"; C "Capacitance (p.u.)"; fbase "Base frequency (Hz)"
      mask init:
      | [iC, iR, omegab, rc_mode] = mask_init_RC(dynamic, R, C, fbase);
      mask TypeOptions dynamic: Dynamic | Static | Static omega
  RL : Subsystem  Variant=on  mask(Line){dynamic=Dynamic, R=Rf, L=Lf, fbase=fb}
      mask prompts: dynamic "Dynamic behavior"; R "Series resistance (p.u.)"; L "Inductance (p.u.)"; fbase "Base frequency (Hz)"
      mask init:
      | [invL, omegab, rl_mode] = mask_init_RL(dynamic, L, fbase);
      mask Help: web('Documentation/RL.html')
      mask TypeOptions dynamic: Static | Dynamic | Static omega
  Real-Imag to Complex : RealImagToComplex
  Relational Operator : RelationalOperator  Operator===  OutDataTypeStr=boolean  ZeroCross=off  RndMeth=Simplest  InputSameDT=off
  Relational Operator1 : RelationalOperator  Operator===  OutDataTypeStr=boolean  ZeroCross=off  RndMeth=Simplest  InputSameDT=off
  Saturation Dynamic : sl_discontinuities/Saturation Dynamic  OutMin=[]  OutMax=[]  OutDataTypeStr=Inherit: Same as second input  OutDataType=fixdt(1, 16)  OutScaling=2^-10  DoSatur=off
  Saturation Dynamic1 : sl_discontinuities/Saturation Dynamic  OutMin=[]  OutMax=[]  OutDataTypeStr=Inherit: Same as second input  OutDataType=fixdt(1, 16)  OutScaling=2^-10  DoSatur=off
  Sum : Sum  Inputs=|+-
  Sum{1..2,6,8} (4 alike) : Sum  Inputs=-+|
  Sum3 : Sum  Inputs=|++
  Sum4 : Sum  Inputs=++|
  Sum5 : Sum  Inputs=|++
  Sum7 : Sum  Inputs=|+-
  Sum9 : Sum  Inputs=|++
  vidref : Outport
  viqref : Outport  Port=2
  wires:
  Memory/1 -> PIv_d/2(In2)
  Memory1/1 -> PIv_q/2(In2)
  Relational Operator1/1 -> Memory1/1
  Sum/1 -> PIv_q/1(In1)
  Relational Operator/1 -> Memory/1
  Sum1/1 -> PIv_d/1(In1)
  Gain1/1 -> Saturation Dynamic/3
  Gain/1 -> Saturation Dynamic1/3
  Divide1/1 -> Saturation Dynamic1/1, Gain/1
  Divide/1 -> Saturation Dynamic/1, Gain1/1
  Abs/1 -> Divide/2, Divide1/2
  Real-Imag to Complex/1 -> Abs/1
  Sum5/1 -> Real-Imag to Complex/2, Saturation Dynamic1/2, Abs1/1, Relational Operator1/1  "ilqref"
  Product/1 -> Sum8/1
  vodref/1 -> Sum1/2  "vodref"
  RC/2(v_q) -> viqref/1, RL/4(v_out_q), Sum/2, Cf/1  "voq"
  [omega] -> Product/2
  Lf1/1 -> Product3/2
  Fi/1 -> Sum4/1
  Sum6/1 -> PIi_d/1(In1)
  voqref/1 -> Sum/1  "voqref"
  Product3/1 -> Sum9/2
  Product2/1 -> Sum3/2
  Cf 1/1 -> Product2/2
  Cf/1 -> Product1/2
  Sum4/1 -> Real-Imag to Complex/1, Saturation Dynamic/2, Abs2/1, Relational Operator/1  "ildref"
  Product1/1 -> Sum2/1
  iod/1 -> RC/2(i_d_out), Fi/1  "iod"
  Sum2/1 -> Sum4/2
  Sum7/1 -> PIi_q/1(In1)
  "Lf "/1 -> Product/1
  Sum3/1 -> Sum5/1
  [omega] -> RC/5(omega), Product3/1  "omega"
  ioq/1 -> RC/4(i_q_out), Fi2/1  "ioq"
  Fi2/1 -> Sum5/2
  PIv_d/1(Out1) -> Sum2/2
  PIv_q/1(Out1) -> Sum3/1
  PIi_d/1(Out1) -> Sum8/2
  PIi_q/1(Out1) -> Sum9/1
  omega/1 -> Product2/1, [omega]  "omega"
  [omega] -> Product1/1
  RC/1(v_d) -> vidref/1, RL/2(v_out_d), Cf 1/1, Sum1/1
  RL/1(id) -> Lf1/1, Sum6/1, RC/1(i_d_in)
  RL/2(iq) -> RC/3(i_q_in), "Lf "/1, Sum7/2
  Sum8/1 -> RL/1(v_in_d)  "vidref"
  Sum9/1 -> RL/3(v_in_q)  "viqref"
  Abs1/1 -> Divide1/1
  Abs2/1 -> Divide/1
  Saturation Dynamic1/1 -> Relational Operator1/2, Sum7/1
  Saturation Dynamic/1 -> Relational Operator/2, Sum6/2

== system lib_IC_GFM/intconv_GFM/VCC/static ==
  vodref : Inport
  voqref : Inport  Port=2
  iod : Inport  Port=3
  ioq : Inport  Port=4
  omega : Inport  Port=5
  Terminator : Terminator
  Terminator1 : Terminator
  Terminator2 : Terminator
  vidref : Outport
  viqref : Outport  Port=2
  wires:
  omega/1 -> Terminator2/1  "ioq"
  ioq/1 -> Terminator1/1  "ioq"
  iod/1 -> Terminator/1  "iod"
  vodref/1 -> vidref/1  "vodref"
  voqref/1 -> viqref/1  "voqref"

== system lib_IC_GFM/intconv_GFM/VI/WOF_d ==
  note: 1) Add Subsystem or Model blocks as valid variant choices.
      | 2) You cannot connect blocks at this level. At simulation, connectivity is automatically
      | determined, based on the active variant and port name matching.
  In1 : Inport
  Active : Subsystem  VariantControl=use_Tf == 1
  Bypass : Subsystem  VariantControl=(default)
  Out1 : Outport

== system lib_IC_GFM/intconv_GFM/VI/WOF_q ==
  note: 1) Add Subsystem or Model blocks as valid variant choices.
      | 2) You cannot connect blocks at this level. At simulation, connectivity is automatically
      | determined, based on the active variant and port name matching.
  In1 : Inport
  Active : Subsystem  VariantControl=use_Tf == 1
  Bypass : Subsystem  VariantControl=(default)
  Out1 : Outport

== system lib_IC_GFM/intconv_GFM/PC/LPF_P/Active ==
  In1 : Inport
  Impl : Subsystem
  Out1 : Outport
  wires:
  Impl/1(P_f) -> Out1/1
  In1/1 -> Impl/1(P)

== system lib_IC_GFM/intconv_GFM/PC/LPF_P/Bypass ==
  In1 : Inport
  Out1 : Outport
  wires:
  In1/1 -> Out1/1

== system lib_IC_GFM/intconv_GFM/PC/LPF_Q/Active ==
  In1 : Inport
  Impl : Subsystem
  Out1 : Outport
  wires:
  Impl/1(Q_f) -> Out1/1
  In1/1 -> Impl/1(Q)

== system lib_IC_GFM/intconv_GFM/PC/LPF_Q/Bypass ==
  In1 : Inport
  Out1 : Outport
  wires:
  In1/1 -> Out1/1

== system lib_IC_GFM/intconv_GFM/VCC/dynamic/RC ==
  note: 1) Add Subsystem or Model blocks as valid variant choices.
      | 2) You cannot connect blocks at this level. At simulation, connectivity is automatically
      | determined, based on the active variant and port name matching.
  i_d_in : Inport
  i_d_out : Inport  Port=2
  i_q_in : Inport  Port=3
  i_q_out : Inport  Port=4
  omega : Inport  Port=5
  dynamic : Subsystem  VariantControl=rc_mode == 1  mask{v_d_0=1}
      mask prompts: v_d_0 "Initial condition for v_d"
  static : Subsystem  VariantControl=rc_mode == 2
  static omega : Subsystem  VariantControl=(default)
  v_d : Outport
  v_q : Outport  Port=2

== system lib_IC_GFM/intconv_GFM/VCC/dynamic/RL ==
  note: 1) Add Subsystem or Model blocks as valid variant choices.
      | 2) You cannot connect blocks at this level. At simulation, connectivity is automatically
      | determined, based on the active variant and port name matching.
  v_in_d : Inport
  v_out_d : Inport  Port=2
  v_in_q : Inport  Port=3
  v_out_q : Inport  Port=4
  dynamic : Subsystem  VariantControl=rl_mode == 1
      settings: PortSchema="{\"entries\":[{\"content\":{\"sides\":[{\"content\":{\"connectorIds\":[\"In1\"]},\"type\":\"ConnectorPlacement.EquallySpacedRectSide\",\"uuid\":\"63966e24-f9e7-4b2d-b456-7f4ea5e3f230\"},{\"content\":{\"connectorIds\":[\"In2\",\"In3\",\"In4\",\"Out1\",\"Out2\"],\"side\":\"RIGHT\"},\"type\":\"ConnectorPlacement.EquallySpacedRectSide\",\"uuid\":\"ded6ef04-52fd-47df-8e49-cf16b827098d\"},{\"content\":{\"connectorIds\":[],\"side\":\"TOP\"},\"type\":\"ConnectorPlacement.EquallySpacedRectSide\",\"uuid\":\"f940a985-fa23-4968-ad44-1d76d0e20c6a\"}]},\"type\":\"ConnectorPlacement.EquallySpacedConnector\",\"uuid\":\"20f61d3c-9af2-4982-98ea-af4910e61c9c\"}],\"packageUris\":[\"http://schema.mathworks.com/mf0/Connector/R2020b\"],\"version\":\"1.0\"}"
  static : Subsystem  VariantControl=rl_mode == 2
  static_omega : Subsystem  VariantControl=(default)
  id : Outport
  iq : Outport  Port=2

== system lib_IC_GFM/intconv_GFM/VCC/dynamic/Subsystem ==
  ref : Inport
  y : Inport  Port=2
  Gain : Gain  Gain=Bext
  Gain1 : Gain  Gain=1./Text
  Gain2 : Gain  Gain=Kext
  Integrator : Integrator  InitialCondition=op_intconv_GFM.VCC_dynamic_Subsystem_Integrator
  Sum : Sum  Inputs=++|
  Sum1 : Sum  Inputs=|+-
  Sum6 : Sum  Inputs=|+-
  Out1 : Outport
  wires:
  Gain2/1 -> Out1/1
  Integrator/1 -> Sum/2
  Gain1/1 -> Integrator/1
  Sum6/1 -> Gain1/1
  Sum1/1 -> Sum/1
  Sum/1 -> Gain2/1
  Gain/1 -> Sum1/1
  ref/1 -> Sum6/1, Gain/1
  y/1 -> Sum6/2, Sum1/2

== system lib_IC_GFM/intconv_GFM/VCC/dynamic/Subsystem1 ==
  ref : Inport
  y : Inport  Port=2
  Gain : Gain  Gain=Bext
  Gain1 : Gain  Gain=1./Text
  Gain2 : Gain  Gain=Kext
  Integrator : Integrator  InitialCondition=op_intconv_GFM.VCC_dynamic_Subsystem1_Integrator
  Sum : Sum  Inputs=++|
  Sum1 : Sum  Inputs=|+-
  Sum6 : Sum  Inputs=|+-
  Out1 : Outport
  wires:
  y/1 -> Sum1/2, Sum6/2
  ref/1 -> Gain/1, Sum6/1
  Gain/1 -> Sum1/1
  Sum/1 -> Gain2/1
  Sum1/1 -> Sum/1
  Sum6/1 -> Gain1/1
  Gain1/1 -> Integrator/1
  Integrator/1 -> Sum/2
  Gain2/1 -> Out1/1

== system lib_IC_GFM/intconv_GFM/VCC/dynamic/Subsystem2 ==
  ref : Inport
  y : Inport  Port=2
  Gain : Gain  Gain=Bint
  Gain1 : Gain  Gain=1./Tint
  Gain2 : Gain  Gain=Kint
  Integrator : Integrator  InitialCondition=op_intconv_GFM.VCC_dynamic_Subsystem2_Integrator
  Sum : Sum  Inputs=++|
  Sum1 : Sum  Inputs=|+-
  Sum6 : Sum  Inputs=|+-
  Out1 : Outport
  wires:
  Gain2/1 -> Out1/1
  Integrator/1 -> Sum/2
  Gain1/1 -> Integrator/1
  Sum6/1 -> Gain1/1
  Sum1/1 -> Sum/1
  Sum/1 -> Gain2/1
  Gain/1 -> Sum1/1
  ref/1 -> Sum6/1, Gain/1
  y/1 -> Sum6/2, Sum1/2

== system lib_IC_GFM/intconv_GFM/VCC/dynamic/Subsystem3 ==
  ref : Inport
  y : Inport  Port=2
  Gain : Gain  Gain=Bint
  Gain1 : Gain  Gain=1./Tint
  Gain2 : Gain  Gain=Kint
  Integrator : Integrator  InitialCondition=op_intconv_GFM.VCC_dynamic_Subsystem3_Integrator
  Sum : Sum  Inputs=++|
  Sum1 : Sum  Inputs=|+-
  Sum6 : Sum  Inputs=|+-
  Out1 : Outport
  wires:
  y/1 -> Sum1/2, Sum6/2
  ref/1 -> Gain/1, Sum6/1
  Gain/1 -> Sum1/1
  Sum/1 -> Gain2/1
  Sum1/1 -> Sum/1
  Sum6/1 -> Gain1/1
  Gain1/1 -> Integrator/1
  Integrator/1 -> Sum/2
  Gain2/1 -> Out1/1

== system lib_IC_GFM/intconv_GFM/VCC/dynamic_VC/RC ==
  note: 1) Add Subsystem or Model blocks as valid variant choices.
      | 2) You cannot connect blocks at this level. At simulation, connectivity is automatically
      | determined, based on the active variant and port name matching.
  i_d_in : Inport
  i_d_out : Inport  Port=2
  i_q_in : Inport  Port=3
  i_q_out : Inport  Port=4
  omega : Inport  Port=5
  dynamic : Subsystem  VariantControl=rc_mode == 1  mask{v_d_0=1}
      mask prompts: v_d_0 "Initial condition for v_d"
  static : Subsystem  VariantControl=rc_mode == 2
  static omega : Subsystem  VariantControl=(default)
  v_d : Outport
  v_q : Outport  Port=2

== system lib_IC_GFM/intconv_GFM/VCC/dynamic_VC/Subsystem ==
  ref : Inport
  y : Inport  Port=2
  Gain : Gain  Gain=Bext
  Gain1 : Gain  Gain=1./Text
  Gain2 : Gain  Gain=Kext
  Integrator : Integrator  InitialCondition=op_intconv_GFM.VCC_dynamic_VC_Subsystem_Integrator
  Sum : Sum  Inputs=++|
  Sum1 : Sum  Inputs=|+-
  Sum6 : Sum  Inputs=|+-
  Out1 : Outport
  wires:
  Gain2/1 -> Out1/1
  Integrator/1 -> Sum/2
  Gain1/1 -> Integrator/1
  Sum6/1 -> Gain1/1
  Sum1/1 -> Sum/1
  Sum/1 -> Gain2/1
  Gain/1 -> Sum1/1
  ref/1 -> Sum6/1, Gain/1
  y/1 -> Sum6/2, Sum1/2

== system lib_IC_GFM/intconv_GFM/VCC/dynamic_VC/Subsystem1 ==
  ref : Inport
  y : Inport  Port=2
  Gain : Gain  Gain=Bext
  Gain1 : Gain  Gain=1./Text
  Gain2 : Gain  Gain=Kext
  Integrator : Integrator  InitialCondition=op_intconv_GFM.VCC_dynamic_VC_Subsystem1_Integrator
  Sum : Sum  Inputs=++|
  Sum1 : Sum  Inputs=|+-
  Sum6 : Sum  Inputs=|+-
  Out1 : Outport
  wires:
  y/1 -> Sum1/2, Sum6/2
  ref/1 -> Gain/1, Sum6/1
  Gain/1 -> Sum1/1
  Sum/1 -> Gain2/1
  Sum1/1 -> Sum/1
  Sum6/1 -> Gain1/1
  Gain1/1 -> Integrator/1
  Integrator/1 -> Sum/2
  Gain2/1 -> Out1/1

== system lib_IC_GFM/intconv_GFM/VCC/dynamic_limiting/PIi_d ==
  In1 : Inport
  Gain : Gain  Gain=Kpc
  Gain1 : Gain  Gain=Kic
  I : Integrator  InitialCondition=op_intconv_GFM.VCC_dynamic_limiting_PIi_d_I
  Sum10 : Sum  Inputs=|++
  Out1 : Outport
  wires:
  I/1 -> Sum10/2
  Gain/1 -> Sum10/1
  Sum10/1 -> Out1/1
  In1/1 -> Gain/1, Gain1/1
  Gain1/1 -> I/1

== system lib_IC_GFM/intconv_GFM/VCC/dynamic_limiting/PIi_q ==
  In1 : Inport
  Gain : Gain  Gain=Kpc
  Gain1 : Gain  Gain=Kic
  I : Integrator  InitialCondition=op_intconv_GFM.VCC_dynamic_limiting_PIi_q_I
  Sum10 : Sum  Inputs=|++
  Out1 : Outport
  wires:
  I/1 -> Sum10/2
  Gain/1 -> Sum10/1
  Sum10/1 -> Out1/1
  In1/1 -> Gain/1, Gain1/1
  Gain1/1 -> I/1

== system lib_IC_GFM/intconv_GFM/VCC/dynamic_limiting/PIv_d ==
  In1 : Inport
  In2 : Inport  Port=2
  Gain : Gain  Gain=Kpv
  Gain1 : Gain  Gain=Kiv
  I : Integrator  InitialCondition=op_intconv_GFM.VCC_dynamic_limiting_PIv_d_I
  Product : Product
  Sum10 : Sum  Inputs=|++
  Out1 : Outport
  wires:
  In2/1 -> Product/2
  Product/1 -> I/1
  I/1 -> Sum10/2
  Gain/1 -> Sum10/1
  Sum10/1 -> Out1/1
  In1/1 -> Gain/1, Gain1/1
  Gain1/1 -> Product/1

== system lib_IC_GFM/intconv_GFM/VCC/dynamic_limiting/PIv_q ==
  In1 : Inport
  In2 : Inport  Port=2
  Gain : Gain  Gain=Kpv
  Gain1 : Gain  Gain=Kiv
  I : Integrator  InitialCondition=op_intconv_GFM.VCC_dynamic_limiting_PIv_q_I
  Product : Product
  Sum10 : Sum  Inputs=|++
  Out1 : Outport
  wires:
  Gain1/1 -> Product/1
  In1/1 -> Gain1/1, Gain/1
  Sum10/1 -> Out1/1
  Gain/1 -> Sum10/1
  I/1 -> Sum10/2
  Product/1 -> I/1
  In2/1 -> Product/2

== system lib_IC_GFM/intconv_GFM/VCC/dynamic_limiting/RC ==
  note: 1) Add Subsystem or Model blocks as valid variant choices.
      | 2) You cannot connect blocks at this level. At simulation, connectivity is automatically
      | determined, based on the active variant and port name matching.
  i_d_in : Inport
  i_d_out : Inport  Port=2
  i_q_in : Inport  Port=3
  i_q_out : Inport  Port=4
  omega : Inport  Port=5
  dynamic : Subsystem  VariantControl=rc_mode == 1  mask{v_d_0=1}
      mask prompts: v_d_0 "Initial condition for v_d"
  static : Subsystem  VariantControl=rc_mode == 2
  static omega : Subsystem  VariantControl=(default)
  v_d : Outport
  v_q : Outport  Port=2

== system lib_IC_GFM/intconv_GFM/VCC/dynamic_limiting/RL ==
  note: 1) Add Subsystem or Model blocks as valid variant choices.
      | 2) You cannot connect blocks at this level. At simulation, connectivity is automatically
      | determined, based on the active variant and port name matching.
  v_in_d : Inport
  v_out_d : Inport  Port=2
  v_in_q : Inport  Port=3
  v_out_q : Inport  Port=4
  dynamic : Subsystem  VariantControl=rl_mode == 1
      settings: PortSchema="{\"entries\":[{\"content\":{\"sides\":[{\"content\":{\"connectorIds\":[\"In1\"]},\"type\":\"ConnectorPlacement.EquallySpacedRectSide\",\"uuid\":\"63966e24-f9e7-4b2d-b456-7f4ea5e3f230\"},{\"content\":{\"connectorIds\":[\"In2\",\"In3\",\"In4\",\"Out1\",\"Out2\"],\"side\":\"RIGHT\"},\"type\":\"ConnectorPlacement.EquallySpacedRectSide\",\"uuid\":\"ded6ef04-52fd-47df-8e49-cf16b827098d\"},{\"content\":{\"connectorIds\":[],\"side\":\"TOP\"},\"type\":\"ConnectorPlacement.EquallySpacedRectSide\",\"uuid\":\"f940a985-fa23-4968-ad44-1d76d0e20c6a\"}]},\"type\":\"ConnectorPlacement.EquallySpacedConnector\",\"uuid\":\"20f61d3c-9af2-4982-98ea-af4910e61c9c\"}],\"packageUris\":[\"http://schema.mathworks.com/mf0/Connector/R2020b\"],\"version\":\"1.0\"}"
  static : Subsystem  VariantControl=rl_mode == 2
  static_omega : Subsystem  VariantControl=(default)
  id : Outport
  iq : Outport  Port=2

== system lib_IC_GFM/intconv_GFM/VI/WOF_d/Active ==
  In1 : Inport
  Impl : Subsystem
  Out1 : Outport
  wires:
  Impl/1(Out1) -> Out1/1
  In1/1 -> Impl/1(In1)

== system lib_IC_GFM/intconv_GFM/VI/WOF_d/Bypass ==
  In1 : Inport
  Out1 : Outport
  wires:
  In1/1 -> Out1/1

== system lib_IC_GFM/intconv_GFM/VI/WOF_q/Active ==
  In1 : Inport
  Impl : Subsystem
  Out1 : Outport
  wires:
  Impl/1(Out1) -> Out1/1
  In1/1 -> Impl/1(In1)

== system lib_IC_GFM/intconv_GFM/VI/WOF_q/Bypass ==
  In1 : Inport
  Out1 : Outport
  wires:
  In1/1 -> Out1/1

== system lib_IC_GFM/intconv_GFM/PC/LPF_P/Active/Impl ==
  P : Inport
  Gain : Gain  Gain=iTf
  I : Integrator  InitialCondition=op_intconv_GFM.PC_LPF_P_Active_Impl_I
  Sum4 : Sum  Inputs=|+-
  P_f : Outport
  wires:
  Gain/1 -> I/1
  Sum4/1 -> Gain/1
  P/1 -> Sum4/1
  I/1 -> P_f/1, Sum4/2

== system lib_IC_GFM/intconv_GFM/PC/LPF_Q/Active/Impl ==
  Q : Inport
  Gain : Gain  Gain=iTf
  I : Integrator  InitialCondition=op_intconv_GFM.PC_LPF_Q_Active_Impl_I
  Sum4 : Sum  Inputs=|+-
  Q_f : Outport
  wires:
  Gain/1 -> I/1
  Q/1 -> Sum4/1
  I/1 -> Q_f/1, Sum4/2
  Sum4/1 -> Gain/1

== system lib_IC_GFM/intconv_GFM/VCC/dynamic/RC/dynamic ==
  omega : Inport
  i_d_in : Inport  Port=2
  i_d_out : Inport  Port=3
  i_q_in : Inport  Port=4
  i_q_out : Inport  Port=5
  Gain1 : Gain  Gain=iR
  Gain2 : Gain  Gain=iR
  Gain3 : Gain  Gain=C
  Gain4 : Gain  Gain=C
  Gain5 : Gain  Gain=iC.*omegab
  Gain6 : Gain  Gain=iC.*omegab
  Product : Product
  Product1 : Product
  Sum10 : Sum  Inputs=|-++
  Sum11 : Sum  Inputs=-+|
  Sum12 : Sum  Inputs=|+-
  Sum13 : Sum  Inputs=-+-|
  vd : Integrator  InitialCondition=op_intconv_GFM.VCC_dynamic_RC_dynamic_vd
  vq : Integrator  InitialCondition=op_intconv_GFM.VCC_dynamic_RC_dynamic_vq
  v_d : Outport
  v_q : Outport  Port=2
  wires:
  i_q_out/1 -> Sum12/2  "iq2"
  i_q_in/1 -> Sum12/1  "iq1"
  i_d_out/1 -> Sum11/1  "id2"
  i_d_in/1 -> Sum11/2  "id1"
  vd/1 -> Gain1/1, v_d/1, Gain4/1  "vd"
  Sum12/1 -> Sum13/2
  Gain5/1 -> vq/1
  Gain1/1 -> Sum10/1
  Sum13/1 -> Gain5/1
  omega/1 -> Product1/2, Product/2  "omega"
  Gain6/1 -> vd/1
  Sum11/1 -> Sum10/2
  Product/1 -> Sum13/1
  Gain2/1 -> Sum13/3
  Gain4/1 -> Product/1
  Product1/1 -> Sum10/3
  vq/1 -> Gain3/1, Gain2/1, v_q/1  "vq"
  Gain3/1 -> Product1/1
  Sum10/1 -> Gain6/1

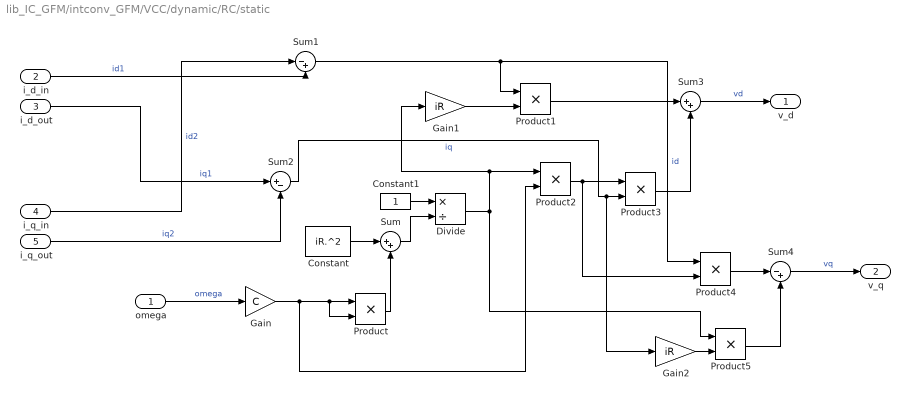
== system lib_IC_GFM/intconv_GFM/VCC/dynamic/RC/static ==
  omega : Inport
  i_d_in : Inport  Port=2
  i_d_out : Inport  Port=3
  i_q_in : Inport  Port=4
  i_q_out : Inport  Port=5
  Constant : Constant  Value=iR.^2
  Constant1 : Constant
  Divide : Product  Inputs=*/
  Gain : Gain  Gain=C
  Gain1 : Gain  Gain=iR
  Gain2 : Gain  Gain=iR
  Product{,1..5} (6 alike) : Product
  Sum : Sum  Inputs=|++
  Sum1 : Sum  Inputs=|-+
  Sum2 : Sum  Inputs=|+-
  Sum3 : Sum  Inputs=|++
  Sum4 : Sum  Inputs=|-+
  v_d : Outport
  v_q : Outport  Port=2
  wires:
  i_q_out/1 -> Sum2/2  "iq2"
  i_d_out/1 -> Sum2/1  "iq1"
  i_q_in/1 -> Sum1/1  "id2"
  i_d_in/1 -> Sum1/2  "id1"
  omega/1 -> Gain/1  "omega"
  Sum3/1 -> v_d/1  "vd"
  Sum4/1 -> v_q/1  "vq"
  Constant/1 -> Sum/1
  Sum/1 -> Divide/2
  Gain/1 -> Product2/2, Product/2, Product/1
  Product/1 -> Sum/2
  Constant1/1 -> Divide/1
  Sum1/1 -> Product1/1, Product4/1  "id"
  Sum2/1 -> Gain2/1, Product3/2  "iq"
  Gain1/1 -> Product1/2
  Divide/1 -> Product5/1, Gain1/1, Product2/1
  Product1/1 -> Sum3/1
  Product3/1 -> Sum3/2
  Product2/1 -> Product4/2, Product3/1
  Product4/1 -> Sum4/1
  Gain2/1 -> Product5/2
  Product5/1 -> Sum4/2
